simulink model "tractor_mu2018"  (R2018a)
settings: Solver=FixedStepDiscrete  StartTime=0.0  StopTime=30  FixedStep=0.001  RelTol=1e-3
model workspace (MAT data in the model file):
  w_2 = Simulink.Parameter
  w_2.DataType = 'auto'
  w_2.Complexity = 'real'
  w_2.Dimensions = [0 0]
undefined symbols (not defined in the file): A, a, B, b, C, D, DiscIntNeverNeededParam, Iz, K, k1, K1, k2, K2, L1, L2, m, magnitude, Phi, Sample_time, Steer_Ratio
libraries: simulink x39, Solver_SF x1, dsparch4 x1
(part 1 of 5)
settings Model: Creator=Lenovo  LastModifiedBy=22872
settings DataIOCC: ReturnWorkspaceOutputs=on
settings SFSimCC: SimUseLocalCustomCode=on
settings RTWCC: RTWUseLocalCustomCode=on

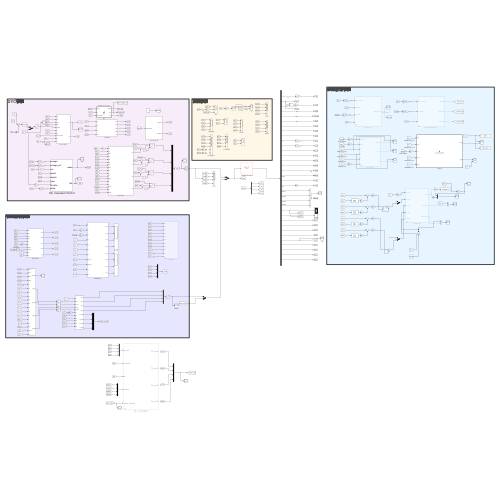
[thumbnail: Simulink's stored preview of the top-level diagram]
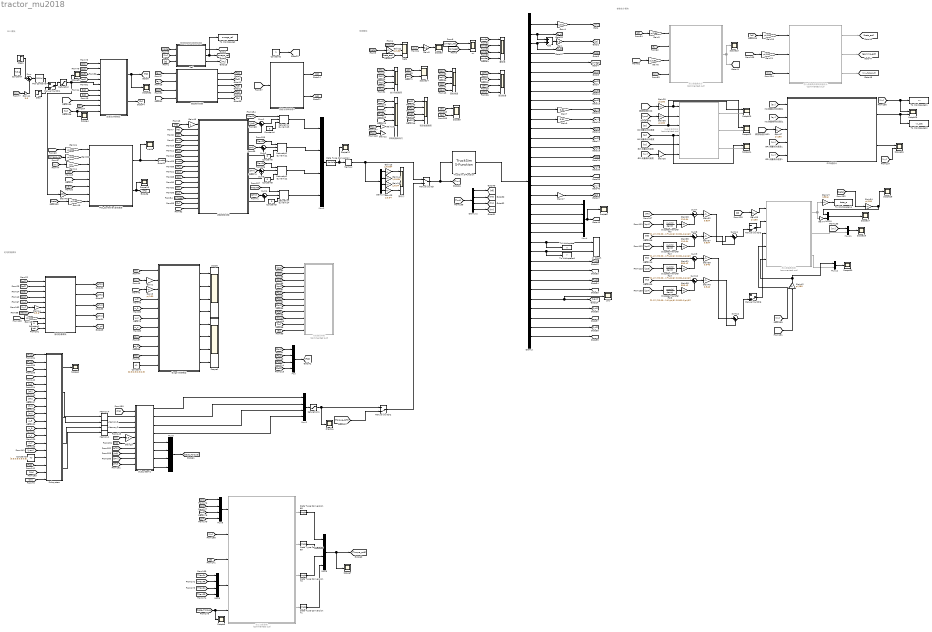
== system tractor_mu2018 ==
  note: 轮地附着模块
  note: 参数估计模块
  note: 观测模块
  note: DYC模块
  note: 理想侧偏角和横摆角速度
  Add : Sum
  Constant : Constant  Value=[0.5;0.5;0.5;0.5]
  Constant{1,4..6,8} (5 alike) : Constant  Value=0
  Constant2 : Constant
  Constant3 : Constant  Value=[0.5;0.5;0.5;0.5]
  Constant7 : Constant  Value=7/3.6
  Data Type Conversion : DataTypeConversion  OutDataTypeStr=double
  Data Type Conversion{68..71} (4 alike) : DataTypeConversion  OutDataTypeStr=single
  Demux : Demux  Outputs=34
  Demux1 : Demux
  Demux2 : Demux
  Discrete Transfer Fcn{,1..3} (4 alike) : DiscreteTransferFcn  Numerator=[2,-2]  Denominator=[(0.001+1/pi/6),(0.001-1/pi/6)]
  Dugoff轮胎模型 : Subsystem
  Gain : Gain  Gain=0.5
  Gain{1..2,26,44} (4 alike) : Gain  Gain=1/3.6
  Gain10 : Gain  Gain=0.5
  Gain{5,11,29,41} (4 alike) : Gain  Gain=3.6
  Gain12 : Gain  Gain=0.5
  Gain13 : Gain  Gain=1/0.834
  Gain14 : Gain  Gain=1/0.834
  Gain15 : Gain  Gain=1/0.94
  Gain17 : Gain  Gain=9.81
  Gain{3,6,8,18..22,24..25,27,30,33..34,36,42} (16 alike) : Gain  Gain=pi/180
  Gain23 : Gain  Gain=1/0.94
  Gain28 : Gain  Gain=110.64
  Gain31 : Gain  Gain=356.42
  Gain32 : Gain  Gain=0.834
  Gain35 : Gain  Gain=110.64
  Gain37 : Gain  Gain=0.834
  Gain38 : Gain  Gain=356.42
  Gain39 : Gain  Gain=0.940
  Gain4 : Gain  Gain=10
  Gain40 : Gain  Gain=0.940
  Gain43 : Gain  Gain=180/pi
  Gain45 : Gain
  Gain46 : Gain  Gain=100
  Gain7 : Gain  Gain=9.81
  Gain9 : Gain  Gain=9.81
  Manual Switch : ManualSwitch
  Manual Switch{1..3,6} (4 alike) : ManualSwitch  CurrentSetting=0
  Memory{,1..4} (5 alike) : Memory
  Mux{,1..5,8..9} (8 alike) : Mux
  Mux10 : Mux  Inputs=2
  Mux11 : Mux  Inputs=2
  Mux12 : Mux  Inputs=2
  PF车速估计 : MATLAB Function  TreatAsAtomicUnit=on  SystemSampleTime=0.01
  PID Controller : simulink/Continuous/PID Controller  Controller=PID  Form=Parallel  TimeDomain=Discrete-time  SampleTime=-1  IntegratorMethod=Forward Euler  FilterMethod=Forward Euler  ControllerParametersSource=internal  P=1.4  I=0.02  D=0  N=100  UseFilter=on  TunerSelectOption=Transfer Function Based (PID Tuner App)  InitialConditionSource=internal  InitialConditionForIntegrator=0  InitialConditionForFilter=0  DifferentiatorICPrevScaledInput=0  ExternalReset=none  TrackingMode=off  Kt=1  LimitOutput=off  UpperSaturationLimit=inf  LowerSaturationLimit=-inf  LinearizeAsGain=on  AntiWindupMode=none  Kb=1  POutMin=[]  POutMax=[]  IOutMin=[]  IOutMax=[]  DOutMin=[]  DOutMax=[]  NOutMin=[]  NOutMax=[]  SumOutMin=[]  SumOutMax=[]  SaturationOutMin=[]  SaturationOutMax=[]  PParamMin=[]  PParamMax=[]  IParamMin=[]  IParamMax=[]  DParamMin=[]  DParamMax=[]  NParamMin=[]  NParamMax=[]  KbParamMin=[]  KbParamMax=[]  KtParamMin=[]  KtParamMax=[]  KbOutMin=[]  KbOutMax=[]  KtOutMin=[]  KtOutMax=[]  IntegratorOutMin=[]  IntegratorOutMax=[]  FilterOutMin=[]  FilterOutMax=[]  SumI1OutMin=[]  SumI1OutMax=[]  SumI2OutMin=[]  SumI2OutMax=[]  SumI3OutMin=[]  SumI3OutMax=[]  SumDOutMin=[]  SumDOutMax=[]  DifferentiatorOutMin=[]  DifferentiatorOutMax=[]  FilterDiffOutCoefMin=[]  FilterDiffOutCoefMax=[]  ReciprocalOutMin=[]  ReciprocalOutMax=[]  SumDenOutMin=[]  SumDenOutMax=[]  SumNumOutMin=[]  SumNumOutMax=[]  DivideOutMin=[]  DivideOutMax=[]  IntegratorContinuousStateAttributes=''  IntegratorStateMustResolveToSignalObject=off  IntegratorRTWStateStorageClass=Auto  FilterContinuousStateAttributes=''  FilterStateMustResolveToSignalObject=off  FilterRTWStateStorageClass=Auto
  PID_Controller/直线循迹 : Subsystem
  Ref : MATLAB Function  TreatAsAtomicUnit=on
  Saturation : Saturate  UpperLimit=1  LowerLimit=0
  Saturation Dynamic{1..4} (4 alike) : simulink/Discontinuities/Saturation Dynamic  OutMin=[]  OutMax=[]  OutDataTypeStr=Inherit: Same as second input  OutDataType=fixdt(1, 16)  OutScaling=2^-10  DoSatur=off
  Saturation1 : Saturate  UpperLimit=9999999  LowerLimit=0
  Scope : Scope  NumInputPorts=4
  Scope1 : Scope  NumInputPorts=4
  Scope{2..4,6..8,12..13,15,27..32} (15 alike) : Scope
  Scope{5,14,22..26} (7 alike) : Scope  NumInputPorts=2
  Step : Step  Time=0  After=0.4  SampleTime=0
  Step1 : Step  Time=0  After=30  SampleTime=0
  Subsystem : Subsystem
  Subsystem1 : Subsystem
  Sum{,7..10} (5 alike) : Sum  Inputs=|+-
  Sum{1..4} (4 alike) : Sum  Inputs=|++  AccumDataTypeStr=single  OutDataTypeStr=single
  Sum11 : Sum  Inputs=|++
  Sum12 : Sum  Inputs=|++
  To Workspace : ToWorkspace  VariableName=X  SaveFormat=Structure  SampleTime=-1
  To Workspace1 : ToWorkspace  VariableName=Y  SaveFormat=Structure  SampleTime=-1
  To Workspace11 : ToWorkspace  VariableName=vx  SaveFormat=Structure With Time  SampleTime=-1
  To Workspace12 : ToWorkspace  VariableName=vx_est  SaveFormat=Structure With Time  SampleTime=-1
  To Workspace14 : ToWorkspace  VariableName=beta_e  SaveFormat=Structure With Time  SampleTime=-1
  To Workspace2 : ToWorkspace  VariableName=omega_ref  SaveFormat=Structure With Time  SampleTime=-1
  TruckSim S-Function : Solver_SF/TruckSim S-Function  Priority=1  SIMFILE=simfile.sim
  XY Graph : simulink/Sinks/XY Graph  xmin=-1  xmax=1  ymin=-1  ymax=1  st=-1
  beta : Scope  NumInputPorts=3
  mode : Scope
  shapley : Scope
  wr : Scope  NumInputPorts=2
  yaw : Scope
  估计车轮载荷 : Scope  NumInputPorts=4
  加速度滑模观测 : Subsystem  Commented=on
  四轮转矩分配 : Subsystem
  四轮转速 : Scope  NumInputPorts=4
  垂直载荷估算 : Subsystem
  实际轮胎纵向力 : Scope  NumInputPorts=6
  实际轮胎载荷 : Scope  NumInputPorts=4
  总驱动力矩制定 : Subsystem
  挡位与刹车处理1 : Subsystem
  滑转率 : Scope  NumInputPorts=4
  质心侧偏角估计 : Subsystem  Commented=on
  质心侧偏角滑模观测器估计 : Subsystem  Commented=on
  质心侧偏角观测 : Subsystem  Commented=on
  车轮腾空判断 : Subsystem  Commented=on
  软土分配策略 : Subsystem  Commented=on
  驱动力 : Scope  NumInputPorts=4
  驱动防滑 : Scope  NumInputPorts=4
  驱动防滑模块 : Subsystem
  wires:
  Demux/1 -> Gain1/1  "Vx"
  Demux/2 -> Add/1, [st_L]  "st_L"
  Demux/3 -> Add/2, [st_R]  "st_R"
  Demux/4 -> [beta]  "deg"
  Demux/5 -> [omega]  "deg/s"
  Add/1 -> Gain/1
  Gain9/1 -> [ay]
  Gain7/1 -> [ax]
  Gain1/1 -> [Vx]
  [Vx] -> Ref/2(vx)
  [mode] -> Ref/1(mode)
  Ref/2(wr_d) -> To Workspace2/1, [omega_ref]
  Ref/1(belta_d) -> [beta_ref]
  [st] -> Ref/3(steer_degree)
  [beta_e] -> beta/1
  [omega_ref] -> wr/1  "omega_ref"
  [beta] -> Gain22/1  "beta"
  [Vx] -> Gain5/1
  [omega] -> wr/2  "omega"
  垂直载荷估算/1(Fz1) -> [Fz1]
  垂直载荷估算/2(Fz2) -> [Fz2]
  垂直载荷估算/3(Fz3) -> [Fz3]
  垂直载荷估算/4(Fz4) -> [Fz4]
  [ax] -> 垂直载荷估算/1(ax)
  [ay] -> 垂直载荷估算/2(ay)
  Demux/6 -> [sp1]  "rpm"
  Demux/7 -> [sp2]
  Demux/8 -> [sp3]
  Demux/9 -> [sp4]
  Demux/10 -> Gain7/1  "g"
  Demux/11 -> Gain9/1  "g"
  Demux/15 -> [FzR2]
  Demux/14 -> [FzR1]
  Demux/13 -> [FzL2]
  Demux/12 -> [FzL1]
  [dTfl] -> 驱动防滑/1
  [dTfr] -> 驱动防滑/2
  [dTrl] -> 驱动防滑/3
  [dTrr] -> 驱动防滑/4
  [Fz1] -> 估计车轮载荷/1
  [Fz2] -> 估计车轮载荷/2
  [Fz3] -> 估计车轮载荷/3
  [Fz4] -> 估计车轮载荷/4
  TruckSim S-Function/1 -> Demux/1
  Mux1/1 -> Data Type Conversion/1
  [sp4] -> 总驱动力矩制定/4(sp4)
  [sp1] -> 总驱动力矩制定/1(sp1)
  [sp3] -> 总驱动力矩制定/3(sp3)
  总驱动力矩制定/1(T0) -> [T0], Scope32/1
  [sp2] -> 总驱动力矩制定/2(sp2)
  [k1] -> 总驱动力矩制定/6(k1)
  [k2] -> 总驱动力矩制定/7(k2)
  [FzR2] -> 四轮转矩分配/7(Fz4)
  [st] -> 四轮转矩分配/3(derta)
  [FzL2] -> 四轮转矩分配/6(Fz3)
  [FzL1] -> 四轮转矩分配/4(Fz1)
  [Mz] -> Gain45/1
  [mode] -> 四轮转矩分配/8(mode)
  [FzR1] -> 四轮转矩分配/5(Fz2)
  [T0] -> 四轮转矩分配/2(T0)
  挡位与刹车处理1/2(spdratio_R) -> [k2]
  挡位与刹车处理1/1(spdratio_F) -> [k1]
  Ref/3(mu) -> [Mu]
  四轮转矩分配/4(Trr) -> Sum4/2
  四轮转矩分配/2(Tfr) -> Sum2/2
  [dTfr] -> Sum2/1
  [dTfl] -> Sum1/1
  四轮转矩分配/1(Tfl) -> Sum1/2
  [dTrl] -> Sum3/1
  四轮转矩分配/3(Trl) -> Sum3/2
  [dTrr] -> Sum4/1
  Demux/16 -> [Roll]  "dRoll"
  Demux/17 -> [dPitch]  "dPitch"
  [Roll] -> 垂直载荷估算/3(roll)
  [Pitch] -> 垂直载荷估算/4(pitch)
  [Vx] -> 质心侧偏角估计/4(vx)
  [ay] -> 质心侧偏角估计/2(Ay_Carsim)
  质心侧偏角估计/1(Beta_estimate_3) -> [beta_e], Scope13/1  "Beta_estimate_3"
  [st] -> Gain3/1
  Gain6/1 -> 质心侧偏角估计/3(Avz_Carsim)
  Gain3/1 -> 质心侧偏角估计/1(Steer_L1_Carsim)
  [omega] -> Gain6/1
  [omega_ref] -> Gain30/1
  PID_Controller/直线循迹/2(Mz) -> Scope15/1, [Mz]
  [omega] -> Gain24/1
  Gain30/1 -> PID_Controller/直线循迹/2(omega_ref)
  Gain24/1 -> PID_Controller/直线循迹/1(omega)
  Step/1 -> Manual Switch1/2
  [beta_est] -> beta/3
  Saturation/1 -> Gain46/1, Scope31/1, 总驱动力矩制定/5(Throttle)
  [sw] -> Scope14/2
  [st] -> Scope14/1
  Demux/19 -> Gain17/1  "XL1"
  [GearD] -> 总驱动力矩制定/8(dTMC_GearD)
  Step1/1 -> Sum/1
  [Vx] -> Gain41/1  "m/s"
  Sum/1 -> PID Controller/1
  Manual Switch1/1 -> Saturation/1
  Gain5/1 -> Scope3/1
  [lamda4] -> 滑转率/4
  [lamda3] -> 滑转率/3
  [lamda2] -> 滑转率/2
  [lamda1] -> 滑转率/1
  [Vx] -> Gain11/1
  Gain11/1 -> PID_Controller/直线循迹/3(vx)
  [dPitch] -> PID_Controller/直线循迹/5(dpitch)
  PID_Controller/直线循迹/1(mode) -> [mode], mode/1
  [k2] -> 四轮转矩分配/11(k2)
  [k1] -> 四轮转矩分配/10(k1)
  [Mu] -> 四轮转矩分配/9(mu)
  Memory/1 -> Manual Switch/1, Demux1/1
  [dPitch] -> 四轮转矩分配/12(dpitch)
  [Vx] -> 四轮转矩分配/13(vx)
  [omega] -> 四轮转矩分配/15(omega)
  总驱动力矩制定/2(Fx) -> [Fx]
  [Fx] -> 四轮转矩分配/16(Fx)
  [Vy] -> 四轮转矩分配/14(vy)
  Gain17/1 -> [az]
  Demux/20 -> Mux4/1  "kappaL1"
  Demux/21 -> Mux4/2  "kappaR1"
  Demux/22 -> Mux4/3  "kappaL2"
  Demux/23 -> Mux4/4  "kappaR2"
  Mux4/1 -> Scope6/1, [kappa]
  [kappa] -> 四轮转矩分配/17(kappa)
  Demux/24 -> To Workspace/1, XY Graph/1
  Demux/25 -> To Workspace1/1, XY Graph/2
  Sum2/1 -> Saturation Dynamic1/2
  Sum3/1 -> Saturation Dynamic2/2
  Sum4/1 -> Saturation Dynamic4/2
  Data Type Conversion/1 -> Scope12/1, Memory/1
  Saturation Dynamic3/1 -> Mux1/1
  Saturation Dynamic1/1 -> Mux1/2
  Saturation Dynamic2/1 -> Mux1/3
  Saturation Dynamic4/1 -> Mux1/4
  PID Controller/1 -> Manual Switch1/1
  Demux/30 -> yaw/1, [yaw]
  Gain/1 -> [st]
  [st] -> PID_Controller/直线循迹/4(derta)
  [yaw] -> PID_Controller/直线循迹/6(yaw)
  Demux/26 -> [FxL1]
  Demux/27 -> [FxR1]
  Demux/28 -> [FxL2]
  Demux/29 -> [FxR2]
  [sp1] -> 车轮腾空判断/1(sp1)
  [sp2] -> 车轮腾空判断/2(sp2)
  [sp3] -> 车轮腾空判断/3(sp3)
  [sp4] -> 车轮腾空判断/4(sp4)
  [FzL1] -> 车轮腾空判断/5(FzL1)
  [FzR1] -> 车轮腾空判断/6(FzR1)
  [FzL2] -> 车轮腾空判断/7(FzL2)
  [FzR2] -> 车轮腾空判断/8(FzR2)
  [Tm4] -> 车轮腾空判断/9(Tm4)
  [Vx] -> 车轮腾空判断/10(vx)  "m/s"
  [az] -> 车轮腾空判断/11(az)  "m/s"
  [beta] -> Gain19/1
  Gain19/1 -> PID_Controller/直线循迹/8(beta)
  Gain21/1 -> 质心侧偏角滑模观测器估计/2(Avz_Carsim)
  质心侧偏角滑模观测器估计/3(vy_hat_out) -> [vy_hat_out]
  质心侧偏角滑模观测器估计/1(beta_est) -> [beta_est]
  质心侧偏角滑模观测器估计/2(gamma_est) -> [gamma_est]
  [Vx] -> 质心侧偏角滑模观测器估计/3(vx)
  [omega] -> Gain21/1
  Gain20/1 -> 质心侧偏角滑模观测器估计/1(Steer_L1_Carsim)
  [st] -> Gain20/1
  Gain22/1 -> beta/2
  [Vx] -> Scope4/1, 总驱动力矩制定/10(vx)  "m/s"
  [vy] -> PF车速估计/5(init_vy)
  [ay] -> PF车速估计/2(ay_m)
  [vy] -> Scope26/2
  PF车速估计/2(vy_est) -> Scope26/1
  PF车速估计/1(vx_est) -> To Workspace12/1, Scope25/2
  [omega] -> Gain27/1
  [ax] -> Scope22/1, 加速度滑模观测/3(ax)
  [vy] -> Gain26/1
  [ax] -> PF车速估计/1(ax_m)
  [Vx] -> PF车速估计/4(init_vx)
  Gain36/1 -> 加速度滑模观测/2(航向角)
  [Vx] -> To Workspace11/1, Scope25/1
  [ay] -> Scope24/1, 加速度滑模观测/4(ay)
  加速度滑模观测/2(ax_c) -> Scope22/2
  [yaw] -> Gain36/1
  加速度滑模观测/1(gamma_c) -> Scope23/2
  [omega] -> Gain25/1
  加速度滑模观测/3(ay_c) -> Scope24/2
  [Vx] -> 加速度滑模观测/5(vx)
  Gain25/1 -> Scope23/1, 加速度滑模观测/1(横摆角速度)
  Gain26/1 -> 加速度滑模观测/6(vy)
  Gain27/1 -> PF车速估计/3(r_m)
  ? -> Manual Switch6/1
  Gain31/1 -> Sum9/2
  Gain40/1 -> Sum12/2
  Gain38/1 -> Sum10/2
  [Trr] -> Sum10/1
  Sum10/1 -> Gain40/1
  Gain32/1 -> Sum11/1
  [sp1] -> Discrete Transfer Fcn/1
  Discrete Transfer Fcn1/1 -> Gain35/1
  Gain37/1 -> Sum11/2
  Sum12/1 -> Manual Switch6/2
  [sp2] -> Discrete Transfer Fcn1/1
  Mux11/1 -> Scope29/1
  [Tfl] -> Sum7/1
  Mux10/1 -> Scope27/1
  Manual Switch3/1 -> 质心侧偏角观测/2(前轮纵向力)
  Sum11/1 -> Manual Switch3/2
  Gain34/1 -> Scope28/1, Mux10/1
  Manual Switch6/1 -> 质心侧偏角观测/3(后轮纵向力)
  Gain39/1 -> Sum12/1
  [Trl] -> Sum9/1
  Gain35/1 -> Sum8/2
  [sp4] -> Discrete Transfer Fcn3/1
  Discrete Transfer Fcn2/1 -> Gain31/1
  Discrete Transfer Fcn3/1 -> Gain38/1
  Discrete Transfer Fcn/1 -> Gain28/1
  质心侧偏角观测/2(纵向速度估计) -> Mux11/2
  Sum8/1 -> Gain37/1
  质心侧偏角观测/3(横摆角速度估计) -> Mux12/2
  Gain33/1 -> 质心侧偏角观测/1(前轮转角)
  Gain42/1 -> Mux12/1, 质心侧偏角观测/5(横摆角速度)
  Sum9/1 -> Gain39/1
  [Vx] -> Mux11/1
  [sp3] -> Discrete Transfer Fcn2/1
  [omega] -> Gain42/1
  [Vx] -> 质心侧偏角观测/4(纵向速度)
  [Tfr] -> Sum8/1
  Mux12/1 -> Scope30/1
  Sum7/1 -> Gain32/1
  质心侧偏角观测/1(侧偏角) -> Gain4/1, Gain43/1  "rad"
  [st] -> Gain33/1
  Gain28/1 -> Sum7/2
  [beta] -> Gain34/1
  Gain43/1 -> To Workspace14/1
  Gain4/1 -> Mux10/2
  Constant2/1 -> [GearD]
  [GearD] -> 挡位与刹车处理1/1(dTMC_GearD)
  [GearD] -> 驱动防滑模块/7(gearD)
  [omega] -> Gain18/1
  [st] -> 驱动防滑模块/10(st)
  Constant1/1 -> 驱动防滑模块/9(brk)
  驱动防滑模块/1(dTfl) -> [dTfl]
  [sp1] -> 驱动防滑模块/1(sp1)
  驱动防滑模块/2(dTfr) -> [dTfr]
  [sp4] -> 驱动防滑模块/4(sp4)
  Gain18/1 -> 驱动防滑模块/8(omega)
  驱动防滑模块/3(dTrl) -> [dTrl]
  驱动防滑模块/4(dTrr) -> [dTrr]
  [sp2] -> 驱动防滑模块/2(sp2)
  [sp3] -> 驱动防滑模块/3(sp3)
  驱动防滑模块/5(v_e) -> [v_e]
  [Vx] -> 驱动防滑模块/5(vx)  "m/s"
  [sp1] -> 四轮转速/1
  [sp2] -> 四轮转速/2
  [sp3] -> 四轮转速/3
  [sp4] -> 四轮转速/4
  [Vx] -> Dugoff轮胎模型/1(vx)  "m/s"
  [vy] -> Gain2/1
  Gain2/1 -> Dugoff轮胎模型/2(vy)
  [omega] -> Gain8/1
  Gain8/1 -> Dugoff轮胎模型/3(wz)
  [w_fl] -> Dugoff轮胎模型/4(w_fl)
  [w_fr] -> Dugoff轮胎模型/5(w_fr)
  [w_rl] -> Dugoff轮胎模型/6(w_rl)
  [w_rr] -> Dugoff轮胎模型/7(w_rr)
  [st_L] -> Dugoff轮胎模型/8(Steer_L1)
  [st_R] -> Dugoff轮胎模型/9(Steer_R1)
  Dugoff轮胎模型/1(Fx_fl) -> Scope/1
  Dugoff轮胎模型/2(Fx_fr) -> Scope/2
  Dugoff轮胎模型/3(Fx_rl) -> Scope/3
  Dugoff轮胎模型/4(Fx_rr) -> Scope/4
  Dugoff轮胎模型/5(Fy_fl) -> Scope1/1
  Dugoff轮胎模型/6(Fy_fr) -> Scope1/2
  Dugoff轮胎模型/7(Fy_rl) -> Scope1/3
  Dugoff轮胎模型/8(Fy_rr) -> Scope1/4
  垂直载荷估算/5(Fz) -> [Fz]
  [Fz0] -> Dugoff轮胎模型/10(Fz)
  Constant/1 -> Dugoff轮胎模型/11(mu)
  [FzL1] -> Mux/1
  [FzL2] -> Mux/2
  [FzR1] -> Mux/3
  [FzR2] -> Mux/4
  Mux/1 -> [Fz0]
  [FxL1] -> 实际轮胎纵向力/1
  [FxR1] -> 实际轮胎纵向力/2
  [FxL2] -> 实际轮胎纵向力/3
  [FxR2] -> 实际轮胎纵向力/4
  [FxL1] -> Subsystem/1(FxL1)
  [w_rr] -> Subsystem/13(wrr)
  [w_rl] -> Subsystem/12(wrl)
  [w_fr] -> Subsystem/11(wfr)
  [w_fl] -> Subsystem/10(wfl)
  [Trr] -> Subsystem/9(Trr)
  [Trl] -> Subsystem/8(Trl)
  [Tfr] -> Subsystem/7(Tfr)
  [Tfl] -> Subsystem/6(Tfl)
  [Vx] -> Subsystem/5(vx)  "m/s"
  [FxR2] -> Subsystem/4(FxR2)
  Subsystem/1(yita_drag) -> Scope2/1
  [yaw] -> Subsystem/14(i)
  Constant3/1 -> Subsystem/15(mu)
  [Fz0] -> Subsystem/16(FZ0)
  [FzR2] -> 实际轮胎载荷/4
  [FzL2] -> 实际轮胎载荷/3
  [FzR1] -> 实际轮胎载荷/2
  [FzL1] -> 实际轮胎载荷/1
  [FxR1] -> Subsystem/3(FxR1)
  [FxL2] -> Subsystem/2(FxL2)
  [FzL1] -> Gain10/1
  [FzL2] -> Gain12/1
  Demux1/1 -> Gain13/1
  Demux1/2 -> Gain14/1
  Demux1/3 -> Gain15/1
  Demux1/4 -> Gain23/1
  Gain13/1 -> 驱动力/1
  Gain14/1 -> 驱动力/2
  Gain15/1 -> 驱动力/3
  Gain23/1 -> 驱动力/4
  Manual Switch/1 -> [Tm4], TruckSim S-Function/1
  Mux2/1 -> Saturation1/1
  [TMaxFL] -> Saturation Dynamic3/1
  [TMaxFR] -> Saturation Dynamic1/1
  Constant6/1 -> Saturation Dynamic1/3
  [TMaxRL] -> Saturation Dynamic2/1
  Constant8/1 -> Saturation Dynamic2/3
  [TMaxRR] -> Saturation Dynamic4/1
  Demux2/1 -> [Tfl]
  Demux2/2 -> [Tfr]
  Demux2/3 -> [Trl]
  Demux2/4 -> [Trr]
  [Tm4] -> Demux2/1
  [T0] -> Subsystem1/1(T0)
  Subsystem/2(phi_FL) -> Memory4/1
  Subsystem/3(phi_FR) -> Memory3/1
  Subsystem/4(phi_RL) -> Memory2/1
  Subsystem/5(phi_RR) -> Memory1/1
  [Vx] -> Gain29/1  "m/s"
  Gain29/1 -> Subsystem1/6(vx)
  [Mz] -> Subsystem1/7(Mz)
  Memory1/1 -> Subsystem1/5(phi_RR)
  Memory2/1 -> Subsystem1/4(phi_RL)
  Memory3/1 -> Subsystem1/3(phi_FR)
  Memory4/1 -> Subsystem1/2(phi_FL)
  Gain41/1 -> Sum/2
  Demux/18 -> [vy]
  [vy] -> Gain44/1
  Gain44/1 -> 驱动防滑模块/6(vy)
  [Mz] -> Subsystem/17(Mz_ref)
  Demux/31 -> [FyL1]
  Demux/32 -> [FyR1]
  Demux/33 -> [FyL2]
  Demux/34 -> [FyR2]
  Saturation1/1 -> shapley/1, Manual Switch2/1
  [dTfl] -> Subsystem1/8(dTfl)
  [dTfr] -> Subsystem1/9(dTfr)
  [dTrl] -> Subsystem1/10(dTrl)
  [dTrr] -> Subsystem1/11(dTrr)
  Subsystem1/1(Tfl_sh) -> Mux2/1
  Subsystem1/2(Tfr_sh) -> Mux2/2
  Subsystem1/3(Trl_sh) -> Mux2/3
  Subsystem1/4(Trr_sh) -> Mux2/4
  [ax] -> 总驱动力矩制定/9(ax)
  [ay] -> Scope5/2
  [ax] -> Scope5/1
  Sum1/1 -> Saturation Dynamic3/2
  Gain45/1 -> 四轮转矩分配/1(Mz)
  软土分配策略/1(Tfl_soft) -> Data Type Conversion68/1
  Mux9/1 -> Scope7/1, [Torque_soft]
  软土分配策略/4(Trr_soft) -> Data Type Conversion71/1
  Data Type Conversion70/1 -> Mux9/3
  Data Type Conversion71/1 -> Mux9/4
  Data Type Conversion69/1 -> Mux9/2
  [sp3] -> Mux8/3
  Mux8/1 -> 软土分配策略/1(sp_all)
  Mux3/1 -> 软土分配策略/4(Tmax)
  [sp4] -> Mux8/4
  软土分配策略/2(Tfr_soft) -> Data Type Conversion69/1
  [st] -> 软土分配策略/3(st)
  软土分配策略/3(Trl_soft) -> Data Type Conversion70/1
  [base_Torque] -> Scope8/1, 软土分配策略/5(base_Torque)
  [Vx] -> 软土分配策略/2(vx(m/s))
  Data Type Conversion68/1 -> Mux9/1
  [sp1] -> Mux8/1
  [sp2] -> Mux8/2
  [TMaxFL] -> Mux3/1
  [TMaxFR] -> Mux3/2
  [TMaxRL] -> Mux3/3
  [TMaxRR] -> Mux3/4
  Subsystem1/5(Tfl_base) -> Mux5/1
  Subsystem1/6(Tfr_base) -> Mux5/2
  Subsystem1/7(Trl_base) -> Mux5/3
  Subsystem1/8(Trr_base) -> Mux5/4
  Mux5/1 -> [base_Torque]
  [Torque_soft] -> Manual Switch2/2
  Manual Switch2/1 -> Manual Switch/2
  Gain46/1 -> PID_Controller/直线循迹/7(throttle)
  Constant4/1 -> Saturation Dynamic3/3
  Constant5/1 -> Saturation Dynamic4/3
  [ax] -> Subsystem/18(ax)

== system tractor_mu2018/Dugoff轮胎模型 ==
  vx : Inport
  vy : Inport  Port=2
  wz : Inport  Port=3
  w_fl : Inport  Port=4
  w_fr : Inport  Port=5
  w_rl : Inport  Port=6
  w_rr : Inport  Port=7
  Steer_L1 : Inport  Port=8
  Steer_R1 : Inport  Port=9
  Fz : Inport  Port=10
  mu : Inport  Port=11
  Demux : Demux
  Gain : Gain  Gain=pi/180
  Gain1 : Gain  Gain=pi/180
  alpha_lamda : Subsystem
  pac2002 : Subsystem
  Fx_fl : Outport
  Fx_fr : Outport  Port=2
  Fx_rl : Outport  Port=3
  Fx_rr : Outport  Port=4
  Fy_fl : Outport  Port=5
  Fy_fr : Outport  Port=6
  Fy_rl : Outport  Port=7
  Fy_rr : Outport  Port=8
  wires:
  Steer_L1/1 -> Gain/1
  vx/1 -> alpha_lamda/1(vx)
  vy/1 -> alpha_lamda/2(vy)
  wz/1 -> alpha_lamda/3(wz)
  w_fl/1 -> alpha_lamda/6(w_fl)
  w_fr/1 -> alpha_lamda/7(w_fr)
  w_rl/1 -> alpha_lamda/8(w_rl)
  w_rr/1 -> alpha_lamda/9(w_rr)
  alpha_lamda/1(lamda_fl) -> pac2002/1(lamda_fl)
  alpha_lamda/2(lamda_fr) -> pac2002/2(lamda_fr)
  alpha_lamda/3(lamda_rl) -> pac2002/3(lamda_rl)
  alpha_lamda/4(lamda_rr) -> pac2002/4(lamda_rr)
  alpha_lamda/5(alpha_fl) -> pac2002/5(alpha_fl)
  alpha_lamda/6(alpha_fr) -> pac2002/6(alpha_fr)
  alpha_lamda/7(alpha_rl) -> pac2002/7(alpha_rl)
  alpha_lamda/8(alpha_rr) -> pac2002/8(alpha_rr)
  Demux/1 -> pac2002/9(Fz_fl)
  Demux/2 -> pac2002/10(Fz_rl)
  Demux/3 -> pac2002/11(Fz_fr)
  Demux/4 -> pac2002/12(Fz_rr)
  pac2002/1(Fx_fl) -> Fx_fl/1
  pac2002/2(Fx_fr) -> Fx_fr/1
  pac2002/3(Fx_rl) -> Fx_rl/1
  pac2002/4(Fx_rr) -> Fx_rr/1
  pac2002/5(Fy_fl) -> Fy_fl/1
  pac2002/6(Fy_fr) -> Fy_fr/1
  pac2002/7(Fy_rl) -> Fy_rl/1
  pac2002/8(Fy_rr) -> Fy_rr/1
  Steer_R1/1 -> Gain1/1
  Gain/1 -> alpha_lamda/4(delta_fl)
  Gain1/1 -> alpha_lamda/5(delta_fr)
  Fz/1 -> Demux/1
  mu/1 -> pac2002/13(mu)

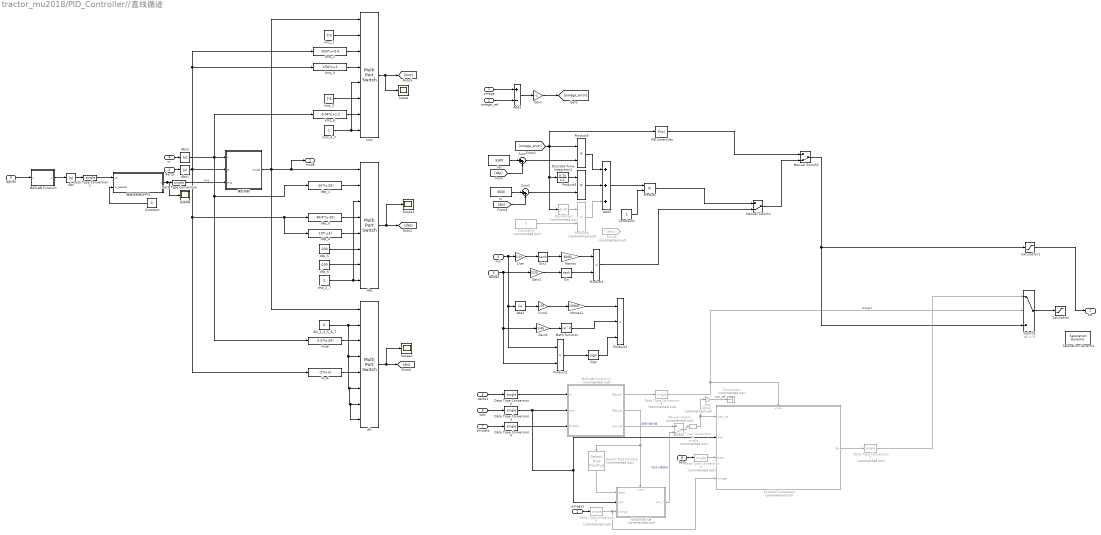
== system tractor_mu2018/PID_Controller//直线循迹 ==
  omega : Inport
  omega_ref : Inport  Port=2
  vx : Inport  Port=3
  derta : Inport  Port=4
  dpitch : Inport  Port=5
  yaw : Inport  Port=6
  throttle : Inport  Port=7
  beta : Inport  Port=8
  1/vm : Gain  Gain=1/10
  1/vm1 : Gain  Gain=1/20
  Abs{,1..3} (4 alike) : Abs
  Add2 : Sum  Inputs=+-
  Add3 : Sum  Inputs=+++
  Constant : Constant  Value=0
  Constant1 : Constant
  Constant5 : Constant  Commented=on  Value=0
  Data Type Conversion{,1..4} (5 alike) : DataTypeConversion  OutDataTypeStr=single
  Data Type Conversion{5..9} (5 alike) : DataTypeConversion  Commented=on  OutDataTypeStr=single
  Derivative1 : Derivative  Commented=on
  Detect Rise Positive : simulink/Logic and Bit Operations/Detect Rise Positive  Commented=on  vinit=0  OutDataTypeStr=boolean
  Discrete-Time Integrator1 : DiscreteIntegrator  SampleTime=-1  ICPrevOutput=DiscIntNeverNeededParam  ICPrevScaledInput=DiscIntNeverNeededParam
  EWMA : Scope
  Enabled Subsystem : Subsystem  Commented=on  TreatAsAtomicUnit=on
  Fcn4 : Fcn  Expr=-2*(u-5)
  Fcn8 : Fcn  Expr=0.5*(u-20)
  From5 : From  Commented=on  GotoTag=kmz
  Gain : Gain  Gain=-1
  Gain1 : Gain  Gain=1/20
  Gain2 : Gain  Gain=1/45
  MATLAB Function : MATLAB Function  TreatAsAtomicUnit=on
  MATLAB Function2 : MATLAB Function  Commented=on  TreatAsAtomicUnit=on
  Manual Switch : ManualSwitch  Commented=on  CurrentSetting=0
  Manual Switch1 : ManualSwitch  CurrentSetting=0
  Manual Switch2 : ManualSwitch  CurrentSetting=0
  Math Function : Math  Operator=magnitude^2  SaturateOnIntegerOverflow=on
  Mzmax : Gain  Gain=8000
  Mzmax1 : Gain  Gain=10000
  PID Controller : simulink/Continuous/PID Controller  Controller=PI  Form=Parallel  TimeDomain=Discrete-time  SampleTime=-1  IntegratorMethod=Forward Euler  FilterMethod=Forward Euler  ControllerParametersSource=internal  P=3000  I=1000  D=0  N=100  UseFilter=on  TunerSelectOption=Transfer Function Based (PID Tuner App)  InitialConditionSource=internal  InitialConditionForIntegrator=0  InitialConditionForFilter=0  DifferentiatorICPrevScaledInput=0  ExternalReset=none  TrackingMode=off  Kt=1  LimitOutput=on  UpperSaturationLimit=inf  LowerSaturationLimit=-inf  LinearizeAsGain=on  AntiWindupMode=back-calculation  Kb=1  POutMin=[]  POutMax=[]  IOutMin=[]  IOutMax=[]  DOutMin=[]  DOutMax=[]  NOutMin=[]  NOutMax=[]  SumOutMin=[]  SumOutMax=[]  SaturationOutMin=[]  SaturationOutMax=[]  PParamMin=[]  PParamMax=[]  IParamMin=[]  IParamMax=[]  DParamMin=[]  DParamMax=[]  NParamMin=[]  NParamMax=[]  KbParamMin=[]  KbParamMax=[]  KtParamMin=[]  KtParamMax=[]  KbOutMin=[]  KbOutMax=[]  KtOutMin=[]  KtOutMax=[]  IntegratorOutMin=[]  IntegratorOutMax=[]  FilterOutMin=[]  FilterOutMax=[]  SumI1OutMin=[]  SumI1OutMax=[]  SumI2OutMin=[]  SumI2OutMax=[]  SumI3OutMin=[]  SumI3OutMax=[]  SumDOutMin=[]  SumDOutMax=[]  DifferentiatorOutMin=[]  DifferentiatorOutMax=[]  FilterDiffOutCoefMin=[]  FilterDiffOutCoefMax=[]  ReciprocalOutMin=[]  ReciprocalOutMax=[]  SumDenOutMin=[]  SumDenOutMax=[]  SumNumOutMin=[]  SumNumOutMax=[]  DivideOutMin=[]  DivideOutMax=[]  IntegratorContinuousStateAttributes=''  IntegratorStateMustResolveToSignalObject=off  IntegratorRTWStateStorageClass=Auto  FilterContinuousStateAttributes=''  FilterStateMustResolveToSignalObject=off  FilterRTWStateStorageClass=Auto
  Product : Product  OutDataTypeStr=single
  Product{1..2,4..5} (4 alike) : Product
  Product3 : Product  Inputs=3
  Product6 : Product  Commented=on
  Saturation : Saturate  UpperLimit=20000  LowerLimit=-20000
  Saturation Dynamic : simulink/Discontinuities/Saturation Dynamic  OutMin=[]  OutMax=[]  OutDataTypeStr=Inherit: Same as second input  OutDataType=fixdt(1, 16)  OutScaling=2^-10  DoSatur=off
  Saturation1 : Saturate  UpperLimit=20000  LowerLimit=-20000
  Scope : Scope
  Scope1 : Scope
  Scope2 : Scope
  Sign : Signum
  Sin : Trigonometry  Operator=tanh
  Sin1 : Trigonometry  Operator=tanh
  Sum : Sum  Inputs=|++
  Sum1 : Sum  Inputs=|++
  Switch1 : Switch  Criteria=u2 > Threshold
  Terminator : Terminator  Commented=on
  deg : Gain  Commented=on  Gain=180/pi
  derta1 : InportShadow  Port=4
  derta2 : InportShadow  Port=4
  dki : MultiPortSwitch  Inputs=7
  dki_1_3_5_6_7 : Constant  Value=0
  dkp : MultiPortSwitch  Inputs=7
  dkp_1 : Fcn  Expr=-10*(u-20)
  dkp_2_7 : Constant  Value=0
  dkp_3 : Fcn  Expr=40/3*(u-10)
  dkp_4 : Fcn  Expr=10*(u-5)
  dkp_5 : Constant  Value=-200
  dkp_6 : Constant  Value=-100
  ki : Constant  Value=3500
  kmz : MultiPortSwitch  Inputs=7
  kmz_1 : Constant  Value=0.9
  kmz_2 : Fcn  Expr=3/50*u+0.6
  kmz_3 : Fcn  Expr=1/50*u+1
  kmz_4_7 : Constant
  kmz_5 : Constant  Value=0.8
  kmz_6 : Fcn  Expr=-0.04*u+1.2
  kp : Constant  Value=5500
  omega1 : InportShadow
  vx1 : InportShadow  Port=3
  指数加权移动平均 : MATLAB Function  TreatAsAtomicUnit=on
  模式判断 : MATLAB Function  TreatAsAtomicUnit=on
  目标航向角计算 : Subsystem  Commented=on  TreatAsAtomicUnit=on
  mode : Outport
  Mz : Outport  Port=2
  wires:
  omega_ref/1 -> Add2/2
  omega/1 -> Add2/1
  Product5/1 -> Add3/1
  Discrete-Time Integrator1/1 -> Product4/1
  [omega_error] -> PID Controller/1, Product5/1, Discrete-Time Integrator1/1, Derivative1/1
  Constant5/1 -> Product6/2
  Product6/1 -> Add3/3
  ki/1 -> Sum1/1
  kp/1 -> Sum/1
  Derivative1/1 -> Product6/1
  Product4/1 -> Add3/2
  Add3/1 -> Product/1
  Add2/1 -> Gain/1
  dpitch/1 -> MATLAB Function/1(u)
  Constant/1 -> 指数加权移动平均/2(is_biased)
  derta/1 -> Abs1/1
  vx/1 -> Abs2/1
  Sum/1 -> Product5/2
  [dkp] -> Sum/2
  Sum1/1 -> Product4/2
  [dki] -> Sum1/2
  模式判断/1(mode) -> kmz/1, dki/1, mode/1, dkp/1
  dkp_2_7/1 -> dkp/3, dkp/8
  dkp_1/1 -> dkp/2
  dkp_3/1 -> dkp/4
  dkp_4/1 -> dkp/5
  dkp_5/1 -> dkp/6
  dkp/1 -> Scope1/1, [dkp]
  Fcn4/1 -> dki/5
  dki/1 -> Scope2/1, [dki]
  kmz/1 -> Scope/1, [kmz]
  kmz_1/1 -> kmz/2
  kmz_2/1 -> kmz/3
  kmz_3/1 -> kmz/4
  kmz_4_7/1 -> kmz/5, kmz/8
  kmz_5/1 -> kmz/6
  kmz_6/1 -> kmz/7
  Fcn8/1 -> dki/3
  dki_1_3_5_6_7/1 -> dki/8, dki/7, dki/6, dki/4, dki/2
  MATLAB Function/1(y) -> Abs/1
  指数加权移动平均/1(y) -> EWMA/1, Data Type Conversion/1
  Abs/1 -> Data Type Conversion1/1
  Abs1/1 -> kmz_3/1, kmz_2/1, dkp_4/1, dkp_3/1, Fcn4/1, 模式判断/2(st)
  Abs2/1 -> kmz_6/1, Fcn8/1, dkp_1/1, 模式判断/1(v)
  dkp_6/1 -> dkp/7
  Gain/1 -> [omega_error]
  Data Type Conversion/1 -> 模式判断/3(avg)  "avg"
  Data Type Conversion1/1 -> 指数加权移动平均/1(uk)
  Enabled Subsystem/1(Mz) -> Data Type Conversion7/1
  Switch1/1 -> Saturation/1
  derta1/1 -> Data Type Conversion2/1
  Data Type Conversion2/1 -> MATLAB Function2/1(st)
  throttle/1 -> Data Type Conversion4/1
  Data Type Conversion4/1 -> MATLAB Function2/3(throttle)
  MATLAB Function2/1(flag_ctrl) -> Data Type Conversion9/1
  MATLAB Function2/3(yaw_ref) -> Manual Switch/1  "直接计算均值"
  MATLAB Function2/2(flag_cnt) -> Detect Rise Positive/1, 目标航向角计算/Enable
  Data Type Conversion3/1 -> MATLAB Function2/2(yaw), 目标航向角计算/2(yaw), Enabled Subsystem/2(yaw)
  omega1/1 -> Data Type Conversion5/1
  Data Type Conversion5/1 -> Enabled Subsystem/4(omega), 目标航向角计算/3(omega)
  目标航向角计算/1(yaw_r) -> Manual Switch/2  "WLS计算目标"
  Manual Switch/1 -> Data Type Conversion8/1
  beta/1 -> Data Type Conversion6/1
  Data Type Conversion6/1 -> Enabled Subsystem/3(beta)
  Manual Switch2/1 -> Switch1/3, Saturation1/1
  yaw/1 -> Data Type Conversion3/1
  Data Type Conversion7/1 -> Switch1/1
  Data Type Conversion8/1 -> Enabled Subsystem/1(yaw_ref), deg/1
  Data Type Conversion9/1 -> Switch1/2, Enabled Subsystem/Enable  "straight"
  deg/1 -> Terminator/1  "yaw_ref"
  Detect Rise Positive/1 -> 目标航向角计算/1(reset)
  Product1/1 -> Manual Switch1/2
  Saturation1/1 -> Mz/1
  vx1/1 -> Product2/1, Abs3/1, 1/vm/1
  1/vm/1 -> Sin1/1
  Mzmax/1 -> Product1/1
  Sin/1 -> Product1/2
  derta2/1 -> Product2/2, Gain2/1, Gain1/1
  Gain1/1 -> Sin/1
  Sin1/1 -> Mzmax/1
  Product/1 -> Manual Switch1/1
  PID Controller/1 -> Manual Switch2/1
  Manual Switch1/1 -> Manual Switch2/2
  1/vm1/1 -> Mzmax1/1
  Gain2/1 -> Math Function/1
  Abs3/1 -> 1/vm1/1
  Product2/1 -> Sign/1
  Mzmax1/1 -> Product3/1
  Math Function/1 -> Product3/2
  Sign/1 -> Product3/3
  Constant1/1 -> Product/2

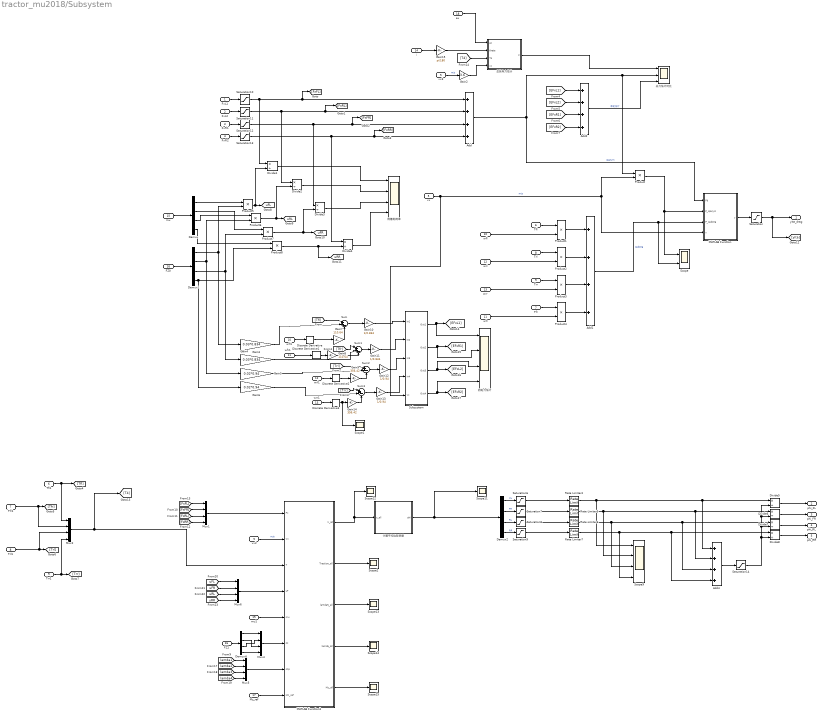
== system tractor_mu2018/Subsystem ==
  FxL1 : Inport
  FxL2 : Inport  Port=2
  FxR1 : Inport  Port=3
  FxR2 : Inport  Port=4
  vx : Inport  Port=5
  Tfl : Inport  Port=6
  Tfr : Inport  Port=7
  Trl : Inport  Port=8
  Trr : Inport  Port=9
  wfl : Inport  Port=10
  wfr : Inport  Port=11
  wrl : Inport  Port=12
  wrr : Inport  Port=13
  i : Inport  Port=14
  mu : Inport  Port=15
  FZ0 : Inport  Port=16
  Mz_ref : Inport  Port=17
  ax : Inport  Port=18
  Add{,1..2,4} (4 alike) : Sum  Inputs=++++
  Demux{,1..2,4} (4 alike) : Demux
  Discrete Derivative{,1..3} (4 alike) : simulink/Discrete/Discrete Derivative  gainval=1.0  ICPrevScaledInput=0.0  OutMin=[]  OutMax=[]  OutDataType=fixdt(1, 16)  OutScaling=2^-10  DoSatur=off
  Divide{1..8} (8 alike) : Product  Inputs=*/
  FZ1 : InportShadow  Port=16
  Gain10 : Gain  Gain=1/0.834
  Gain11 : Gain  Gain=1/0.834
  Gain12 : Gain  Gain=1/0.94
  Gain13 : Gain  Gain=1/0.94
  Gain14 : Gain  Gain=356.42
  Gain15 : Gain  Gain=pi/180
  Gain2 : Gain  Gain=3.6
  Gain3 : Gain  Gain=0.03*0.834
  Gain4 : Gain  Gain=0.03*0.834
  Gain5 : Gain  Gain=0.02*0.94
  Gain6 : Gain  Gain=0.02*0.94
  Gain7 : Gain  Gain=110.64
  Gain8 : Gain  Gain=110.64
  Gain9 : Gain  Gain=356.42
  MATLAB Function : MATLAB Function  TreatAsAtomicUnit=on
  MATLAB Function3 : MATLAB Function  TreatAsAtomicUnit=on
  Mux{1..2,4..6} (5 alike) : Mux
  Product{,1..8} (9 alike) : Product
  Rate Limiter{4..7} (4 alike) : RateLimiter  RisingSlewLimit=2e5  FallingSlewLimit=-2e5  SampleTimeMode=inherited
  Saturation : Saturate  UpperLimit=999  LowerLimit=-999
  Saturation{6..13} (8 alike) : Saturate  UpperLimit=99999999  LowerLimit=0
  Saturation14 : Saturate  UpperLimit=99999999999999  LowerLimit=0.01
  Scope : Scope  NumInputPorts=2
  Scope{1..2,11..15} (7 alike) : Scope
  Scope9 : Scope  NumInputPorts=4
  Subsystem : Subsystem
  Sum{,1..3} (4 alike) : Sum  Inputs=|+--
  Tfl1 : InportShadow  Port=6
  Tfr1 : InportShadow  Port=7
  Trl1 : InportShadow  Port=8
  Trr1 : InportShadow  Port=9
  mu1 : InportShadow  Port=15
  vx2 : InportShadow  Port=5
  vx3 : InportShadow  Port=5
  wfl1 : InportShadow  Port=10
  wfr1 : InportShadow  Port=11
  wrl1 : InportShadow  Port=12
  wrr1 : InportShadow  Port=13
  四轮力估计 : Scope  NumInputPorts=4
  总力估计对比 : Scope  NumInputPorts=3
  总纵向力估计 : Subsystem
  计算平均边际贡献 : MATLAB Function  TreatAsAtomicUnit=on
  附着利用率 : Scope  NumInputPorts=4
  yita_drag : Outport
  phi_FL : Outport  Port=2
  phi_FR : Outport  Port=3
  phi_RL : Outport  Port=4
  phi_RR : Outport  Port=5
  tag scope: uFL=global, uFR=global, uRL=global, uRR=global
  wires:
  FxR2/1 -> Saturation13/1
  FxR1/1 -> Saturation12/1
  FxL2/1 -> Saturation11/1
  FxL1/1 -> Saturation10/1
  Tfl/1 -> Product1/1
  wfl/1 -> Product1/2
  Trl/1 -> Product2/1
  Trr/1 -> Product3/1
  wrr/1 -> Product3/2
  wrl/1 -> Product2/2
  wfr/1 -> Product4/2
  Tfr/1 -> Product4/1
  Product4/1 -> Add1/4
  Product3/1 -> Add1/3
  Product2/1 -> Add1/2
  Product1/1 -> Add1/1
  Add1/1 -> MATLAB Function/3(P_qudong), Scope/2  "qudong"
  MATLAB Function/1(y) -> Saturation/1
  Add/1 -> Product/1, 总力估计对比/2, MATLAB Function/1(Fd)  "qianyin"
  vx/1 -> MATLAB Function/4(v), Product/2, Subsystem/5(vx)  "m/s"
  Product/1 -> Scope/1, MATLAB Function/2(P_qianyin)
  mu/1 -> Demux/1
  FZ0/1 -> Demux1/1
  Demux/1 -> Product5/1
  Product5/1 -> [uFL], Divide1/2
  Demux/2 -> Product7/1
  Product6/1 -> [uRL], Divide2/2
  Demux/3 -> Product6/1
  Demux/4 -> Product8/1
  Product7/1 -> [uFR], Divide3/2
  Product8/1 -> [uRR], Divide4/2
  Saturation/1 -> [yita], yita_drag/1
  Divide2/1 -> 附着利用率/2
  Divide1/1 -> 附着利用率/1
  Divide4/1 -> 附着利用率/4
  Divide3/1 -> 附着利用率/3
  计算平均边际贡献/1(phi) -> Demux2/1, Scope11/1
  Demux2/2 -> Saturation7/1  "FR"
  Demux2/1 -> Saturation6/1  "FL"
  Demux2/3 -> Saturation8/1  "RL"
  Demux2/4 -> Saturation9/1  "RR"
  Rate Limiter4/1 -> Scope9/1, Divide5/1, Add4/1
  Rate Limiter5/1 -> Scope9/2, Add4/2, Divide6/1
  Rate Limiter6/1 -> Scope9/3, Divide7/1, Add4/3
  Add4/1 -> Saturation14/1
  Divide5/1 -> phi_FL/1
  Divide6/1 -> phi_FR/1
  Divide7/1 -> phi_RL/1
  Divide8/1 -> phi_RR/1
  Mux1/1 -> MATLAB Function3/1(Fx)
  vx2/1 -> MATLAB Function3/2(Vx)  "m/s"
  Tfl1/1 -> [Tfl], Mux2/1
  Tfr1/1 -> [Tfr], Mux2/2
  Trr1/1 -> [Trr], Mux2/4
  mu1/1 -> MATLAB Function3/5(mu)
  FZ1/1 -> Demux4/1
  Demux4/1 -> Mux4/1
  Demux4/4 -> Mux4/4
  Demux4/2 -> Mux4/3
  Demux4/3 -> Mux4/2
  Mux4/1 -> MATLAB Function3/6(Fz)
  Mz_ref/1 -> MATLAB Function3/8(Mz_ref)
  MATLAB Function3/1(V_all) -> Scope12/1, 计算平均边际贡献/1(v_all)
  MATLAB Function3/2(Traction_all) -> Scope2/1
  MATLAB Function3/3(lamdaN_all) -> Scope13/1
  MATLAB Function3/4(lamda_all) -> Scope14/1
  MATLAB Function3/5(Mz_all) -> Scope15/1
  Saturation10/1 -> [FxFL], Add/1, Divide1/1
  Saturation11/1 -> [FxRL], Add/2, Divide2/1
  Saturation12/1 -> [FxFR], Add/3, Divide3/1
  Saturation13/1 -> [FxRR], Add/4, Divide4/1
  Saturation6/1 -> Rate Limiter4/1
  Saturation7/1 -> Rate Limiter5/1
  Saturation8/1 -> Rate Limiter6/1
  Saturation9/1 -> Rate Limiter7/1
  Rate Limiter7/1 -> Scope9/4, Add4/4, Divide8/1
  Saturation14/1 -> Divide8/2, Divide7/2, Divide6/2, Divide5/2
  Mux5/1 -> MATLAB Function3/7(slip)
  [lamda1] -> Mux5/1
  [lamda2] -> Mux5/2
  [lamda3] -> Mux5/3
  [lamda4] -> Mux5/4
  [uRR] -> Mux6/4
  [uRL] -> Mux6/3
  [uFR] -> Mux6/2
  [uFL] -> Mux6/1
  Mux6/1 -> MATLAB Function3/4(uF)
  [FxRR] -> Mux1/4
  [FxRL] -> Mux1/3
  [FxFR] -> Mux1/2
  [FxFL] -> Mux1/1
  ax/1 -> 总纵向力估计/1(ax)
  Mux2/1 -> [T4], MATLAB Function3/3(T)
  [T4] -> 总纵向力估计/3(T4)
  vx3/1 -> Gain2/1  "m/s"
  Gain2/1 -> 总纵向力估计/4(vx)
  Gain15/1 -> 总纵向力估计/2(theta)
  总纵向力估计/1(F) -> 总力估计对比/1
  Gain12/1 -> Subsystem/3(In3)
  Gain11/1 -> Subsystem/2(In2)
  Demux1/1 -> Gain3/1, Product5/2
  Gain10/1 -> Subsystem/1(In1)
  [Trr] -> Sum3/1
  Sum3/1 -> Gain13/1
  Gain5/1 -> Sum2/2
  [Tfr] -> Sum1/1
  [Trl] -> Sum2/1
  wrl1/1 -> Discrete Derivative2/1
  Sum/1 -> Gain10/1
  wrr1/1 -> Discrete Derivative3/1
  Discrete Derivative2/1 -> Gain9/1
  Sum1/1 -> Gain11/1
  Gain4/1 -> Sum1/2
  Gain6/1 -> Sum3/2
  [Tfl] -> Sum/1
  wfl1/1 -> Discrete Derivative/1
  Sum2/1 -> Gain12/1
  Gain8/1 -> Sum1/3
  Discrete Derivative1/1 -> Gain8/1
  Gain7/1 -> Sum/3
  Discrete Derivative/1 -> Gain7/1
  Gain3/1 -> Sum/2
  Gain14/1 -> Sum3/3
  Demux1/3 -> Gain4/1, Product7/2
  Demux1/2 -> Product6/2, Gain5/1
  Demux1/4 -> Gain6/1, Product8/2
  Gain9/1 -> Sum2/3
  wfr1/1 -> Discrete Derivative1/1
  Trl1/1 -> [Trl], Mux2/3
  i/1 -> Gain15/1
  [EFxL1] -> Add2/1
  [EFxL2] -> Add2/2
  [EFxR1] -> Add2/3
  [EFxR2] -> Add2/4
  Add2/1 -> 总力估计对比/3  "单轮估计"
  Discrete Derivative3/1 -> Scope1/1, Gain14/1
  Subsystem/1(Out1) -> 四轮力估计/1, [EFxL1]
  Subsystem/2(Out2) -> 四轮力估计/2, [EFxR1]
  Subsystem/3(Out3) -> 四轮力估计/3, [EFxL2]
  Gain13/1 -> Subsystem/4(In4)
  Subsystem/4(Out4) -> 四轮力估计/4, [EFxR2]

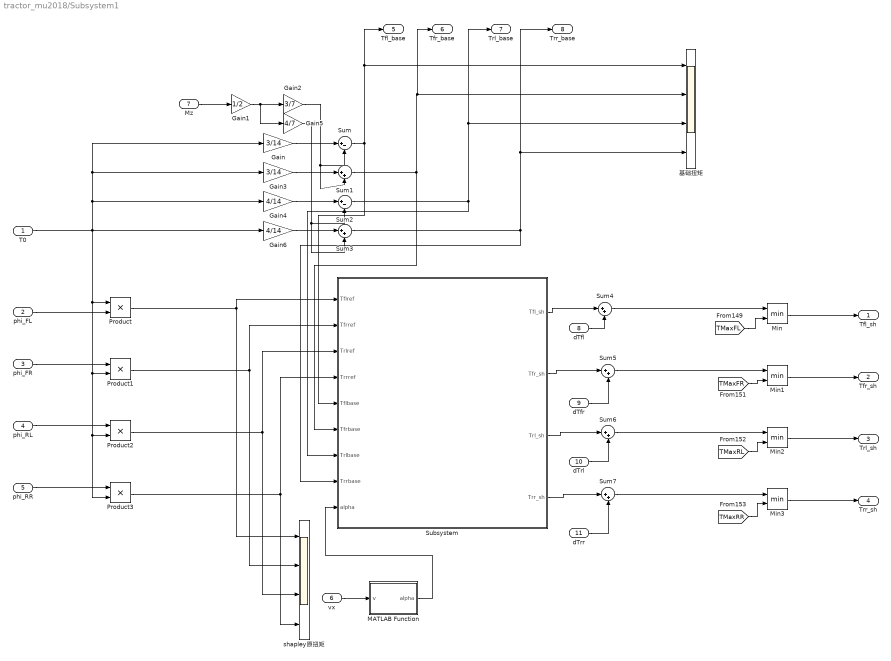
== system tractor_mu2018/Subsystem1 ==
  T0 : Inport
  phi_FL : Inport  Port=2
  phi_FR : Inport  Port=3
  phi_RL : Inport  Port=4
  phi_RR : Inport  Port=5
  vx : Inport  Port=6
  Mz : Inport  Port=7
  dTfl : Inport  Port=8
  dTfr : Inport  Port=9
  dTrl : Inport  Port=10
  dTrr : Inport  Port=11
  Gain : Gain  Gain=3/14
  Gain1 : Gain  Gain=1/2
  Gain2 : Gain  Gain=3/7
  Gain3 : Gain  Gain=3/14
  Gain4 : Gain  Gain=4/14
  Gain5 : Gain  Gain=4/7
  Gain6 : Gain  Gain=4/14
  MATLAB Function : MATLAB Function  TreatAsAtomicUnit=on
  Min{,1..3} (4 alike) : MinMax  Inputs=2
  Product{,1..3} (4 alike) : Product
  Subsystem : Subsystem
  Sum : Sum  Inputs=|+-
  Sum{1,3..7} (6 alike) : Sum  Inputs=|++
  Sum2 : Sum  Inputs=|+-
  shapley原扭矩 : Scope  NumInputPorts=4
  基础扭矩 : Scope  NumInputPorts=4
  Tfl_sh : Outport
  Tfr_sh : Outport  Port=2
  Trl_sh : Outport  Port=3
  Trr_sh : Outport  Port=4
  Tfl_base : Outport  Port=5
  Tfr_base : Outport  Port=6
  Trl_base : Outport  Port=7
  Trr_base : Outport  Port=8
  wires:
  phi_RR/1 -> Product3/1
  [TMaxFR] -> Min1/2
  phi_FR/1 -> Product1/1
  T0/1 -> Product3/2, Product2/2, Product1/2, Product/1, Gain6/1, Gain4/1, Gain3/1, Gain/1
  [TMaxRR] -> Min3/2
  phi_FL/1 -> Product/2
  [TMaxFL] -> Min/2
  [TMaxRL] -> Min2/2
  phi_RL/1 -> Product2/1
  Gain/1 -> Sum/1
  Mz/1 -> Gain1/1
  Gain1/1 -> Gain5/1, Gain2/1
  Gain2/1 -> Sum1/2, Sum/2
  Gain3/1 -> Sum1/1
  Gain4/1 -> Sum2/1
  Gain5/1 -> Sum3/2, Sum2/2
  Gain6/1 -> Sum3/1
  Sum/1 -> Subsystem/5(Tflbase), Tfl_base/1, 基础扭矩/1
  Sum1/1 -> Subsystem/6(Tfrbase), Tfr_base/1, 基础扭矩/2
  Sum2/1 -> Subsystem/7(Trlbase), Trl_base/1, 基础扭矩/3
  Sum3/1 -> Subsystem/8(Trrbase), Trr_base/1, 基础扭矩/4
  vx/1 -> MATLAB Function/1(v)
  MATLAB Function/1(alpha) -> Subsystem/9(alpha)
  Product/1 -> shapley原扭矩/1, Subsystem/1(Tflref)
  Product1/1 -> shapley原扭矩/2, Subsystem/2(Tfrref)
  Product2/1 -> shapley原扭矩/3, Subsystem/3(Trlref)
  Product3/1 -> shapley原扭矩/4, Subsystem/4(Trrref)
  Subsystem/1(Tfl_sh) -> Sum4/1
  Subsystem/2(Tfr_sh) -> Sum5/1
  Subsystem/3(Trl_sh) -> Sum6/1
  Subsystem/4(Trr_sh) -> Sum7/1
  Min/1 -> Tfl_sh/1
  Min1/1 -> Tfr_sh/1
  Min2/1 -> Trl_sh/1
  Min3/1 -> Trr_sh/1
  dTfl/1 -> Sum4/2
  Sum4/1 -> Min/1
  dTfr/1 -> Sum5/2
  Sum5/1 -> Min1/1
  dTrl/1 -> Sum6/2
  Sum6/1 -> Min2/1
  dTrr/1 -> Sum7/2
  Sum7/1 -> Min3/1

== system tractor_mu2018/加速度滑模观测 ==
  横摆角速度 : Inport
  航向角 : Inport  Port=2
  ax : Inport  Port=3
  ay : Inport  Port=4
  vx : Inport  Port=5
  vy : Inport  Port=6
  Constant : Constant  Value=0
  MATLAB Function : MATLAB Function  TreatAsAtomicUnit=on
  MATLAB Function1 : MATLAB Function  TreatAsAtomicUnit=on
  Pulse Generator : DiscretePulseGenerator  PulseType=Time based  Period=0.05  PulseWidth=2
  gamma_c : Outport
  ax_c : Outport  Port=2
  ay_c : Outport  Port=3
  wires:
  横摆角速度/1 -> MATLAB Function/1(gamma_m)
  航向角/1 -> MATLAB Function/2(phi_GPS)
  MATLAB Function/2(gamma_corrected) -> MATLAB Function1/5(gamma_c), gamma_c/1
  Pulse Generator/1 -> MATLAB Function1/6(GPS_update_flag), MATLAB Function/3(GPS_valid)
  ax/1 -> MATLAB Function1/1(a_xm)
  ay/1 -> MATLAB Function1/2(a_ym)
  vx/1 -> MATLAB Function1/3(v_xGPS)
  vy/1 -> MATLAB Function1/4(v_yGPS)
  MATLAB Function1/2(a_yc) -> ay_c/1
  MATLAB Function1/1(a_xc) -> ax_c/1
  Constant/1 -> MATLAB Function1/7(reset)

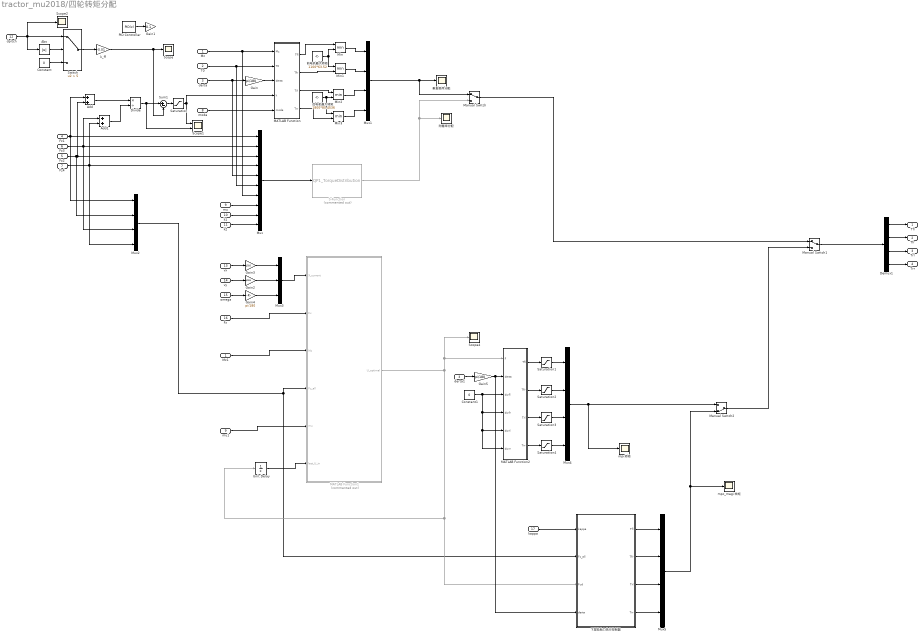
== system tractor_mu2018/四轮转矩分配 ==
  Mz : Inport
  T0 : Inport  Port=2
  derta : Inport  Port=3
  Fz1 : Inport  Port=4
  Fz2 : Inport  Port=5
  Fz3 : Inport  Port=6
  Fz4 : Inport  Port=7
  mode : Inport  Port=8
  mu : Inport  Port=9
  k1 : Inport  Port=10
  k2 : Inport  Port=11
  dpitch : Inport  Port=12
  vx : Inport  Port=13
  vy : Inport  Port=14
  omega : Inport  Port=15
  Fx : Inport  Port=16
  kappa : Inport  Port=17
  Abs : Abs
  Add : Sum
  Add1 : Sum
  Constant : Constant  Value=0
  Constant1 : Constant  Value=0
  Demux1 : Demux
  Divide : Product  Inputs=*/
  Gain : Gain  Gain=pi/180
  Gain1 : Gain  Gain=0.1
  Gain2 : Gain  Gain=1/3.6
  Gain3 : Gain  Gain=1/3.6
  Gain4 : Gain  Gain=pi/180
  Gain5 : Gain  Gain=pi/180
  MATLAB Function : MATLAB Function  TreatAsAtomicUnit=on
  MATLAB Function1 : MATLAB Function  Commented=on  TreatAsAtomicUnit=on
  MATLAB Function2 : MATLAB Function  TreatAsAtomicUnit=on
  Manual Switch : ManualSwitch
  Manual Switch1 : ManualSwitch
  Manual Switch2 : ManualSwitch  CurrentSetting=0
  Min{,1..3} (4 alike) : MinMax  Inputs=2
  Mux : Mux  Inputs=10
  Mux{1..2,4..5} (4 alike) : Mux
  Mux3 : Mux  Inputs=3
  Mz1 : InportShadow
  PID Controller : simulink/Continuous/PID Controller  Controller=PID  Form=Parallel  TimeDomain=Discrete-time  SampleTime=-1  IntegratorMethod=Forward Euler  FilterMethod=Forward Euler  ControllerParametersSource=internal  P=3  I=1  D=0  N=100  UseFilter=on  TunerSelectOption=Transfer Function Based (PID Tuner App)  InitialConditionSource=internal  InitialConditionForIntegrator=0  InitialConditionForFilter=0  DifferentiatorICPrevScaledInput=0  ExternalReset=none  TrackingMode=off  Kt=1  LimitOutput=off  UpperSaturationLimit=inf  LowerSaturationLimit=-inf  LinearizeAsGain=on  AntiWindupMode=none  Kb=1  POutMin=[]  POutMax=[]  IOutMin=[]  IOutMax=[]  DOutMin=[]  DOutMax=[]  NOutMin=[]  NOutMax=[]  SumOutMin=[]  SumOutMax=[]  SaturationOutMin=[]  SaturationOutMax=[]  PParamMin=[]  PParamMax=[]  IParamMin=[]  IParamMax=[]  DParamMin=[]  DParamMax=[]  NParamMin=[]  NParamMax=[]  KbParamMin=[]  KbParamMax=[]  KtParamMin=[]  KtParamMax=[]  KbOutMin=[]  KbOutMax=[]  KtOutMin=[]  KtOutMax=[]  IntegratorOutMin=[]  IntegratorOutMax=[]  FilterOutMin=[]  FilterOutMax=[]  SumI1OutMin=[]  SumI1OutMax=[]  SumI2OutMin=[]  SumI2OutMax=[]  SumI3OutMin=[]  SumI3OutMax=[]  SumDOutMin=[]  SumDOutMax=[]  DifferentiatorOutMin=[]  DifferentiatorOutMax=[]  FilterDiffOutCoefMin=[]  FilterDiffOutCoefMax=[]  ReciprocalOutMin=[]  ReciprocalOutMax=[]  SumDenOutMin=[]  SumDenOutMax=[]  SumNumOutMin=[]  SumNumOutMax=[]  DivideOutMin=[]  DivideOutMax=[]  IntegratorContinuousStateAttributes=''  IntegratorStateMustResolveToSignalObject=off  IntegratorRTWStateStorageClass=Auto  FilterContinuousStateAttributes=''  FilterStateMustResolveToSignalObject=off  FilterRTWStateStorageClass=Auto
  S-Function : S-Function  Commented=on  FunctionName=QP1_TorqueDistribution  SFunctionDeploymentMode=off  EnableBusSupport=off
  Saturation : Saturate  UpperLimit=1  LowerLimit=0.3
  Saturation1 : Saturate  UpperLimit=1100*63.52  LowerLimit=0
  Saturation2 : Saturate  UpperLimit=1100*63.52  LowerLimit=0
  Saturation3 : Saturate  UpperLimit=1800*80.4  LowerLimit=0
  Saturation4 : Saturate  UpperLimit=1800*80.4  LowerLimit=0
  Scope : Scope
  Scope1 : Scope  NumInputPorts=2
  Scope2 : Scope
  Scope4 : Scope
  Sum1 : Sum  Inputs=|+-
  Switch : Switch  Criteria=u2 > Threshold  Threshold=5
  Unit Delay : UnitDelay  SampleTime=-1  HasFrameUpgradeWarning=on
  derta1 : InportShadow  Port=3
  k_ff : Gain  Gain=-0.01
  mpc_magic转矩 : Scope
  mpc转矩 : Scope
  mu1 : InportShadow  Port=9
  下层轮胎力执行控制器 : Subsystem
  前电机最大转矩 : Constant  Value=1100*63.52
  后电机最大转矩 : Constant  Value=1800*80.4536
  垂直载荷分配 : Scope
  附着率分配 : Scope
  Tfl : Outport
  Tfr : Outport  Port=2
  Trl : Outport  Port=3
  Trr : Outport  Port=4
  wires:
  T0/1 -> MATLAB Function/2(T0), Mux/6
  Fz1/1 -> Mux2/1, Mux/1, Add/1
  Fz2/1 -> Mux2/2, Add/2, Mux/3
  Fz3/1 -> Mux2/3, Add1/1, Mux/2
  Fz4/1 -> Add1/2, Mux/4, Mux2/4
  derta/1 -> Gain/1, Mux/5
  mode/1 -> MATLAB Function/5(mode)
  MATLAB Function/1(Tfl) -> Min/1
  前电机最大转矩/1 -> Min1/1, Min/2
  MATLAB Function/2(Tfr) -> Min1/2
  MATLAB Function/3(Trl) -> Min2/1
  后电机最大转矩/1 -> Min3/1, Min2/2
  MATLAB Function/4(Trr) -> Min3/2
  Mux/1 -> S-Function/1
  mu/1 -> Mux/8
  k1/1 -> Mux/9
  k2/1 -> Mux/10
  S-Function/1 -> 附着率分配/1, Manual Switch/2
  Demux1/1 -> Tfl/1
  Demux1/2 -> Tfr/1
  Demux1/3 -> Trl/1
  Demux1/4 -> Trr/1
  Manual Switch/1 -> Manual Switch1/1
  Min/1 -> Mux1/1
  Min1/1 -> Mux1/2
  Min2/1 -> Mux1/3
  Min3/1 -> Mux1/4
  Mux1/1 -> 垂直载荷分配/1, Manual Switch/1
  Add/1 -> Divide/1
  Add1/1 -> Divide/2
  PID Controller/1 -> Gain1/1
  Sum1/1 -> Saturation/1
  dpitch/1 -> Scope2/1, Abs/1, Switch/1
  Divide/1 -> Scope1/2, Sum1/1
  Abs/1 -> Switch/2
  Constant/1 -> Switch/3
  Switch/1 -> k_ff/1
  k_ff/1 -> Scope/1, Sum1/2
  Saturation/1 -> Scope1/1, MATLAB Function/4(k)
  Mz1/1 -> MATLAB Function1/3(Mz)
  Mux2/1 -> 下层轮胎力执行控制器/2(Fz_all), MATLAB Function1/4(Fz_all)
  mu1/1 -> MATLAB Function1/5(mu)
  omega/1 -> Gain4/1
  vy/1 -> Gain2/1
  vx/1 -> Gain3/1
  Mux3/1 -> MATLAB Function1/1(X_current)
  Unit Delay/1 -> MATLAB Function1/6(last_U_in)
  MATLAB Function1/1(U_optimal) -> 下层轮胎力执行控制器/3(Fud), Unit Delay/1, Scope4/1, MATLAB Function2/1(F)
  Fx/1 -> MATLAB Function1/2(Fx)
  Gain2/1 -> Mux3/2
  Gain3/1 -> Mux3/1
  Gain4/1 -> Mux3/3
  Gain/1 -> MATLAB Function/3(derta)
  derta1/1 -> Gain5/1
  Gain5/1 -> 下层轮胎力执行控制器/4(derta), MATLAB Function2/2(derta)
  MATLAB Function2/4(Trr) -> Saturation4/1
  MATLAB Function2/3(Trl) -> Saturation3/1
  MATLAB Function2/2(Tfr) -> Saturation2/1
  MATLAB Function2/1(Tfl) -> Saturation1/1
  Mux4/1 -> mpc转矩/1, Manual Switch2/1
  Manual Switch1/1 -> Demux1/1
  Saturation1/1 -> Mux4/1
  Saturation2/1 -> Mux4/2
  Saturation3/1 -> Mux4/3
  Saturation4/1 -> Mux4/4
  Constant1/1 -> MATLAB Function2/6(dwrr), MATLAB Function2/5(dwrl), MATLAB Function2/4(dwfr), MATLAB Function2/3(dwfl)
  kappa/1 -> 下层轮胎力执行控制器/1(kappa)
  下层轮胎力执行控制器/1(Tfl) -> Mux5/1
  下层轮胎力执行控制器/2(Tfr) -> Mux5/2
  下层轮胎力执行控制器/3(Trl) -> Mux5/3
  下层轮胎力执行控制器/4(Trr) -> Mux5/4
  Mux5/1 -> mpc_magic转矩/1, Manual Switch2/2
  Manual Switch2/1 -> Manual Switch1/2
  Mz/1 -> Mux/7, MATLAB Function/1(Mz)

== system tractor_mu2018/垂直载荷估算 ==
  ax : Inport
  ay : Inport  Port=2
  roll : Inport  Port=3
  pitch : Inport  Port=4
  MATLAB Function : MATLAB Function  TreatAsAtomicUnit=on
  MATLAB Function1 : MATLAB Function  Commented=on  TreatAsAtomicUnit=on
  MATLAB Function2 : MATLAB Function  Commented=on  TreatAsAtomicUnit=on
  Mux : Mux
  axay : Scope  Commented=on  NumInputPorts=4
  原方法 : Scope  Commented=on  NumInputPorts=4
  Fz1 : Outport
  Fz2 : Outport  Port=2
  Fz3 : Outport  Port=3
  Fz4 : Outport  Port=4
  Fz : Outport  Port=5
  wires:
  ax/1 -> MATLAB Function2/1(ax), MATLAB Function1/1(ax), MATLAB Function/1(ax)
  ay/1 -> MATLAB Function2/2(ay), MATLAB Function1/2(ay), MATLAB Function/2(ay)
  MATLAB Function/2(Fz2) -> Mux/2, Fz2/1
  MATLAB Function/3(Fz3) -> Mux/3, Fz3/1
  MATLAB Function/4(Fz4) -> Mux/4, Fz4/1
  pitch/1 -> MATLAB Function2/3(alpha), MATLAB Function1/3(alpha), MATLAB Function/3(alpha)
  roll/1 -> MATLAB Function2/4(belta), MATLAB Function1/4(belta), MATLAB Function/4(belta)
  MATLAB Function1/1(Fz1) -> axay/1
  MATLAB Function1/2(Fz2) -> axay/2
  MATLAB Function1/3(Fz3) -> axay/3
  MATLAB Function1/4(Fz4) -> axay/4
  MATLAB Function2/1(Fz1) -> 原方法/1
  MATLAB Function2/2(Fz2) -> 原方法/2
  MATLAB Function2/3(Fz3) -> 原方法/3
  MATLAB Function2/4(Fz4) -> 原方法/4
  MATLAB Function/1(Fz1) -> Mux/1, Fz1/1
  Mux/1 -> Fz/1
